simulink model "sys1"  (R2023b)
settings: Solver=VariableStepAuto  StartTime=0.0  StopTime=30e-3  RelTol=1e-3
InitFcn:
  | fs = 100e6;
  | ts = 1 / fs;
values from neighbouring files (symbols this model uses):
  c = 3e8    (= 300000000)    [init_param.m]
  H_az1 = zeros(numSamples,numPulses)    [init_param.m]
  H_az2 = zeros(numSamples,numPulses)    [init_param.m]
  H_ref = fft(conj(fliplr(txChirp)), numSamples)    [init_param.m]
  rawData = rawData + 0.01 * (randn(size(rawData)) + 1j * randn(size(rawData)))    [init_param.m]
  x1 = zeros(size(rawData))    [main.m]
  x2 = zeros(size(x1))    [main.m]
  x3 = zeros(size(x2))    [main.m]
  x4 = zeros(size(x3))    [main.m]
  x5 = zeros(size(x4))    [main.m]
  x6 = zeros(size(x5))    [main.m]
  xx4 = zeros(size(xx3))    [main.m]
  xx5 = zeros(size(xx4))    [main.m]
  xx6 = zeros(size(xx5))    [main.m]
undefined symbols (not defined in the file or in its folder): ffva1156, w2, w3, w4, w5, w6, w7, w8, w9, ww2, ww3, ww4, ww5, ww6, ww7, ww8, ww9, xcku095
libraries: hdlBasic x917, hdlDSPIP x18, dspsrcs4 x12, vmcUtilities x1
(part 4 of 9)

== system sys1/SAR/stream/stream_ifft/stage6 ==
  en : Inport
  re : Inport  Port=2
  im : Inport  Port=3
  BF : Subsystem
      settings: PortSchema="{\"entries\":[{\"content\":{\"sides\":[{\"content\":{\"connectorIds\":[\"In1\",\"In2\",\"Out3\",\"Out4\",\"In3\",\"In4\"]},\"type\":\"ConnectorPlacement.EquallySpacedRectSide\",\"uuid\":\"975bd1ab-81ed-4ae7-b1e2-8f492a85d8f1\"},{\"content\":{\"connectorIds\":[\"Out1\",\"Out2\"],\"side\":\"RIGHT\"},\"type\":\"ConnectorPlacement.EquallySpacedRectSide\",\"uuid\":\"1eadf147-5ad8-47d9-8b00-0d3bf9cf32a8\"},{\"content\":{\"side\":\"TOP\"},\"type\":\"ConnectorPlacement.EquallySpacedRectSide\",\"uuid\":\"8c547c25-4f14-4718-a05d-45e4b8488b96\"}]},\"type\":\"ConnectorPlacement.EquallySpacedConnector\",\"uuid\":\"01bb5c7b-b675-4632-bc6b-a159d4a2e208\"}],\"packageUris\":[\"http://schema.mathworks.com/mf0/Connector/R2020b\"],\"version\":\"1.0\"}"
  Constant : hdlBasic/Constant  const=2^15  gui_display_data_type=Fixed-point  arith_type=Unsigned  n_bits=20  bin_pt=0  preci_type=Single  exp_width=8  frac_width=24  explicit_period=off  period=1  XmcBlockStatus=1  maskContainerNames=tabcontainer1  block_type=constant  block_config=sysgen:Constant_config
  Constant1 : hdlBasic/Constant  const=1  gui_display_data_type=Boolean  arith_type=Boolean  n_bits=16  bin_pt=14  preci_type=Single  exp_width=8  frac_width=24  explicit_period=on  period=ts  XmcBlockStatus=1  maskContainerNames=tabcontainer1  block_type=constant  block_config=sysgen:Constant_config
  Counter1 : hdlBasic/Counter  cnt_type=Free running  cnt_to=Inf  operation=Up  start_count=0  cnt_by_val=1  arith_type=Unsigned  n_bits=20  bin_pt=0  load_pin=off  rst=off  en=on  explicit_period=Explicit  period=ts  use_behavioral_HDL=off  implementation=Fabric  XmcBlockStatus=1  maskContainerNames=group1  block_type=counter  block_config=sysgen:Counter_config  block_width=531  block_height=1023
  Delay11 : hdlBasic/Delay  rst=off  en=off  latency=6  reg_retiming=off  XmcBlockStatus=1  maskContainerNames=group1  block_type=delay  block_config=sysgen:Delay_config
  Delay7 : hdlBasic/Delay  rst=off  en=off  latency=1  reg_retiming=off  XmcBlockStatus=1  maskContainerNames=group1  block_type=delay  block_config=sysgen:Delay_config
  Delay8 : hdlBasic/Delay  rst=off  en=off  latency=1  reg_retiming=off  XmcBlockStatus=1  maskContainerNames=group1  block_type=delay  block_config=sysgen:Delay_config
  Multiplexer : Subsystem
      settings: PortSchema="{\"entries\":[{\"content\":{\"sides\":[{\"content\":{\"connectorIds\":[\"In1\",\"In2\",\"In3\",\"In4\"]},\"type\":\"ConnectorPlacement.EquallySpacedRectSide\",\"uuid\":\"d39b2674-e61f-4632-a918-ea673b128ff5\"},{\"content\":{\"connectorIds\":[\"Out1\",\"Out2\"],\"side\":\"RIGHT\"},\"type\":\"ConnectorPlacement.EquallySpacedRectSide\",\"uuid\":\"03c9bc0a-e0d2-45eb-9b7a-9d06bc1b3e13\"},{\"content\":{\"connectorIds\":[\"In5\"],\"side\":\"TOP\"},\"type\":\"ConnectorPlacement.EquallySpacedRectSide\",\"uuid\":\"49e788e0-ebb0-431e-96ea-edf312796710\"}]},\"type\":\"ConnectorPlacement.EquallySpacedConnector\",\"uuid\":\"eef61444-07bb-4ce5-a4f8-b8563d493c59\"}],\"packageUris\":[\"http://schema.mathworks.com/mf0/Connector/R2020b\"],\"version\":\"1.0\"}"
  Register2 : hdlBasic/Register  init=0  rst=off  en=on  XmcBlockStatus=1  maskContainerNames=tabcontainer1  block_type=register  block_config=sysgen:Register_config
  Relational : hdlBasic/Relational  mode=a=b  op_type=Bool  en=off  latency=0  XmcBlockStatus=1  maskContainerNames=tabcontainer1  block_type=relational  block_config=sysgen:Relational_config
  Shift2 : hdlBasic/Shift  shift_dir=Right  shift_bits=1  en=off  latency=0  precision=User Defined  arith_type="Signed  (2's comp)"  n_bits=16  bin_pt=0  quantization="Round  (unbiased: +/- Inf)"  overflow=Flag as error  XmcBlockStatus=1  maskContainerNames=group2  block_type=shift  block_config=sysgen:Shift_config
  Shift3 : hdlBasic/Shift  shift_dir=Right  shift_bits=1  en=off  latency=0  precision=User Defined  arith_type="Signed  (2's comp)"  n_bits=16  bin_pt=0  quantization="Round  (unbiased: +/- Inf)"  overflow=Flag as error  XmcBlockStatus=1  maskContainerNames=group2  block_type=shift  block_config=sysgen:Shift_config
  Twiddle1 : Subsystem
      settings: PortSchema="{\"entries\":[{\"content\":{\"sides\":[{\"content\":{\"connectorIds\":[\"In1\",\"In2\"]},\"type\":\"ConnectorPlacement.EquallySpacedRectSide\",\"uuid\":\"3a95ef15-fc61-4ad6-8380-7417c0bf925f\"},{\"content\":{\"connectorIds\":[\"Out1\",\"Out2\"],\"side\":\"RIGHT\"},\"type\":\"ConnectorPlacement.EquallySpacedRectSide\",\"uuid\":\"0430fa0d-aaaf-45a9-9ba5-469212780f48\"},{\"content\":{\"connectorIds\":[\"In3\"],\"side\":\"TOP\"},\"type\":\"ConnectorPlacement.EquallySpacedRectSide\",\"uuid\":\"c44a7ed1-335c-4ec2-97d7-9de8a0fe1bfa\"}]},\"type\":\"ConnectorPlacement.EquallySpacedConnector\",\"uuid\":\"1391f0d5-c6a7-4a7e-8f95-f600f2d41ad0\"}],\"packageUris\":[\"http://schema.mathworks.com/mf0/Connector/R2020b\"],\"version\":\"1.0\"}"
  delay : Subsystem
      settings: PortSchema="{\"entries\":[{\"content\":{\"sides\":[{\"content\":{\"connectorIds\":[\"In1\",\"In2\"]},\"type\":\"ConnectorPlacement.EquallySpacedRectSide\",\"uuid\":\"8e95d830-f739-4680-8e8d-a694a3d776c9\"},{\"content\":{\"connectorIds\":[\"Out1\",\"Out2\",\"In4\",\"In5\"],\"side\":\"RIGHT\"},\"type\":\"ConnectorPlacement.EquallySpacedRectSide\",\"uuid\":\"bd1208a8-56cb-479f-9e66-9cf6d0e57587\"},{\"content\":{\"connectorIds\":[\"In3\"],\"side\":\"TOP\"},\"type\":\"ConnectorPlacement.EquallySpacedRectSide\",\"uuid\":\"57cbc148-baa9-4a2d-b86c-5e5c9d420efc\"}]},\"type\":\"ConnectorPlacement.EquallySpacedConnector\",\"uuid\":\"451ef570-de0a-4096-83a7-e8ad0739923f\"}],\"packageUris\":[\"http://schema.mathworks.com/mf0/Connector/R2020b\"],\"version\":\"1.0\"}"
  valid : Outport
  out_re : Outport  Port=2
  out_im : Outport  Port=3
  wires:
  Shift3/1 -> Delay8/1
  Shift2/1 -> Delay7/1
  Constant1/1 -> Register2/1
  Relational/1 -> Register2/2
  Constant/1 -> Relational/2
  re/1 -> Shift2/1
  im/1 -> Shift3/1
  Register2/1 -> Delay11/1
  Counter1/1 -> Multiplexer/5(cnt), Twiddle1/3(cnt), delay/3(cnt), Relational/1
  BF/1(Out2_r) -> Multiplexer/3(r1)
  BF/2(Out2_i) -> Multiplexer/4(i1)
  Twiddle1/2(ii) -> BF/4(vi)
  Twiddle1/1(rr) -> BF/3(vr)
  BF/3(Out1_r) -> delay/4(r1)
  BF/4(Out1_i) -> delay/5(i1)
  delay/1(rr) -> Multiplexer/1(r2), BF/1(ur)
  delay/2(ii) -> Multiplexer/2(i2), BF/2(ui)
  Delay7/1 -> delay/1(r), Twiddle1/1(r)
  Delay8/1 -> delay/2(i), Twiddle1/2(i)
  en/1 -> Counter1/1
  Delay11/1 -> valid/1
  Multiplexer/1(rr) -> out_re/1
  Multiplexer/2(ii) -> out_im/1

== system sys1/SAR/stream/stream_ifft/stage7 ==
  en : Inport
  re : Inport  Port=2
  im : Inport  Port=3
  BF : Subsystem
      settings: PortSchema="{\"entries\":[{\"content\":{\"sides\":[{\"content\":{\"connectorIds\":[\"In1\",\"In2\",\"Out3\",\"Out4\",\"In3\",\"In4\"]},\"type\":\"ConnectorPlacement.EquallySpacedRectSide\",\"uuid\":\"975bd1ab-81ed-4ae7-b1e2-8f492a85d8f1\"},{\"content\":{\"connectorIds\":[\"Out1\",\"Out2\"],\"side\":\"RIGHT\"},\"type\":\"ConnectorPlacement.EquallySpacedRectSide\",\"uuid\":\"1eadf147-5ad8-47d9-8b00-0d3bf9cf32a8\"},{\"content\":{\"side\":\"TOP\"},\"type\":\"ConnectorPlacement.EquallySpacedRectSide\",\"uuid\":\"8c547c25-4f14-4718-a05d-45e4b8488b96\"}]},\"type\":\"ConnectorPlacement.EquallySpacedConnector\",\"uuid\":\"01bb5c7b-b675-4632-bc6b-a159d4a2e208\"}],\"packageUris\":[\"http://schema.mathworks.com/mf0/Connector/R2020b\"],\"version\":\"1.0\"}"
  Constant : hdlBasic/Constant  const=2^16  gui_display_data_type=Fixed-point  arith_type=Unsigned  n_bits=20  bin_pt=0  preci_type=Single  exp_width=8  frac_width=24  explicit_period=off  period=1  XmcBlockStatus=1  maskContainerNames=tabcontainer1  block_type=constant  block_config=sysgen:Constant_config
  Constant1 : hdlBasic/Constant  const=1  gui_display_data_type=Boolean  arith_type=Boolean  n_bits=16  bin_pt=14  preci_type=Single  exp_width=8  frac_width=24  explicit_period=on  period=ts  XmcBlockStatus=1  maskContainerNames=tabcontainer1  block_type=constant  block_config=sysgen:Constant_config
  Counter1 : hdlBasic/Counter  cnt_type=Free running  cnt_to=Inf  operation=Up  start_count=0  cnt_by_val=1  arith_type=Unsigned  n_bits=20  bin_pt=0  load_pin=off  rst=off  en=on  explicit_period=Explicit  period=ts  use_behavioral_HDL=off  implementation=Fabric  XmcBlockStatus=1  maskContainerNames=group1  block_type=counter  block_config=sysgen:Counter_config  block_width=531  block_height=1023
  Delay11 : hdlBasic/Delay  rst=off  en=off  latency=6  reg_retiming=off  XmcBlockStatus=1  maskContainerNames=group1  block_type=delay  block_config=sysgen:Delay_config
  Delay7 : hdlBasic/Delay  rst=off  en=off  latency=1  reg_retiming=off  XmcBlockStatus=1  maskContainerNames=group1  block_type=delay  block_config=sysgen:Delay_config
  Delay8 : hdlBasic/Delay  rst=off  en=off  latency=1  reg_retiming=off  XmcBlockStatus=1  maskContainerNames=group1  block_type=delay  block_config=sysgen:Delay_config
  Multiplexer : Subsystem
      settings: PortSchema="{\"entries\":[{\"content\":{\"sides\":[{\"content\":{\"connectorIds\":[\"In1\",\"In2\",\"In3\",\"In4\"]},\"type\":\"ConnectorPlacement.EquallySpacedRectSide\",\"uuid\":\"d39b2674-e61f-4632-a918-ea673b128ff5\"},{\"content\":{\"connectorIds\":[\"Out1\",\"Out2\"],\"side\":\"RIGHT\"},\"type\":\"ConnectorPlacement.EquallySpacedRectSide\",\"uuid\":\"03c9bc0a-e0d2-45eb-9b7a-9d06bc1b3e13\"},{\"content\":{\"connectorIds\":[\"In5\"],\"side\":\"TOP\"},\"type\":\"ConnectorPlacement.EquallySpacedRectSide\",\"uuid\":\"49e788e0-ebb0-431e-96ea-edf312796710\"}]},\"type\":\"ConnectorPlacement.EquallySpacedConnector\",\"uuid\":\"eef61444-07bb-4ce5-a4f8-b8563d493c59\"}],\"packageUris\":[\"http://schema.mathworks.com/mf0/Connector/R2020b\"],\"version\":\"1.0\"}"
  Register2 : hdlBasic/Register  init=0  rst=off  en=on  XmcBlockStatus=1  maskContainerNames=tabcontainer1  block_type=register  block_config=sysgen:Register_config
  Relational : hdlBasic/Relational  mode=a=b  op_type=Bool  en=off  latency=0  XmcBlockStatus=1  maskContainerNames=tabcontainer1  block_type=relational  block_config=sysgen:Relational_config
  Shift2 : hdlBasic/Shift  shift_dir=Right  shift_bits=1  en=off  latency=0  precision=User Defined  arith_type="Signed  (2's comp)"  n_bits=16  bin_pt=0  quantization="Round  (unbiased: +/- Inf)"  overflow=Flag as error  XmcBlockStatus=1  maskContainerNames=group2  block_type=shift  block_config=sysgen:Shift_config
  Shift3 : hdlBasic/Shift  shift_dir=Right  shift_bits=1  en=off  latency=0  precision=User Defined  arith_type="Signed  (2's comp)"  n_bits=16  bin_pt=0  quantization="Round  (unbiased: +/- Inf)"  overflow=Flag as error  XmcBlockStatus=1  maskContainerNames=group2  block_type=shift  block_config=sysgen:Shift_config
  Twiddle1 : Subsystem
      settings: PortSchema="{\"entries\":[{\"content\":{\"sides\":[{\"content\":{\"connectorIds\":[\"In1\",\"In2\"]},\"type\":\"ConnectorPlacement.EquallySpacedRectSide\",\"uuid\":\"3a95ef15-fc61-4ad6-8380-7417c0bf925f\"},{\"content\":{\"connectorIds\":[\"Out1\",\"Out2\"],\"side\":\"RIGHT\"},\"type\":\"ConnectorPlacement.EquallySpacedRectSide\",\"uuid\":\"0430fa0d-aaaf-45a9-9ba5-469212780f48\"},{\"content\":{\"connectorIds\":[\"In3\"],\"side\":\"TOP\"},\"type\":\"ConnectorPlacement.EquallySpacedRectSide\",\"uuid\":\"c44a7ed1-335c-4ec2-97d7-9de8a0fe1bfa\"}]},\"type\":\"ConnectorPlacement.EquallySpacedConnector\",\"uuid\":\"1391f0d5-c6a7-4a7e-8f95-f600f2d41ad0\"}],\"packageUris\":[\"http://schema.mathworks.com/mf0/Connector/R2020b\"],\"version\":\"1.0\"}"
  delay : Subsystem
      settings: PortSchema="{\"entries\":[{\"content\":{\"sides\":[{\"content\":{\"connectorIds\":[\"In1\",\"In2\"]},\"type\":\"ConnectorPlacement.EquallySpacedRectSide\",\"uuid\":\"8e95d830-f739-4680-8e8d-a694a3d776c9\"},{\"content\":{\"connectorIds\":[\"Out1\",\"Out2\",\"In4\",\"In5\"],\"side\":\"RIGHT\"},\"type\":\"ConnectorPlacement.EquallySpacedRectSide\",\"uuid\":\"bd1208a8-56cb-479f-9e66-9cf6d0e57587\"},{\"content\":{\"connectorIds\":[\"In3\"],\"side\":\"TOP\"},\"type\":\"ConnectorPlacement.EquallySpacedRectSide\",\"uuid\":\"57cbc148-baa9-4a2d-b86c-5e5c9d420efc\"}]},\"type\":\"ConnectorPlacement.EquallySpacedConnector\",\"uuid\":\"451ef570-de0a-4096-83a7-e8ad0739923f\"}],\"packageUris\":[\"http://schema.mathworks.com/mf0/Connector/R2020b\"],\"version\":\"1.0\"}"
  valid : Outport
  out_re : Outport  Port=2
  out_im : Outport  Port=3
  wires:
  Shift3/1 -> Delay8/1
  Shift2/1 -> Delay7/1
  Delay11/1 -> valid/1
  en/1 -> Counter1/1
  Delay8/1 -> Twiddle1/2(i), delay/2(i)
  Delay7/1 -> Twiddle1/1(r), delay/1(r)
  delay/2(ii) -> Multiplexer/2(i2), BF/2(ui)
  delay/1(rr) -> Multiplexer/1(r2), BF/1(ur)
  BF/4(Out1_i) -> delay/5(i1)
  BF/3(Out1_r) -> delay/4(r1)
  Twiddle1/1(rr) -> BF/3(vr)
  Twiddle1/2(ii) -> BF/4(vi)
  BF/2(Out2_i) -> Multiplexer/4(i1)
  BF/1(Out2_r) -> Multiplexer/3(r1)
  Counter1/1 -> Relational/1, delay/3(cnt), Twiddle1/3(cnt), Multiplexer/5(cnt)
  Register2/1 -> Delay11/1
  im/1 -> Shift3/1
  re/1 -> Shift2/1
  Constant/1 -> Relational/2
  Relational/1 -> Register2/2
  Constant1/1 -> Register2/1
  Multiplexer/1(rr) -> out_re/1
  Multiplexer/2(ii) -> out_im/1

== system sys1/SAR/stream/stream_ifft/stage8 ==
  en : Inport
  re : Inport  Port=2
  im : Inport  Port=3
  BF : Subsystem
      settings: PortSchema="{\"entries\":[{\"content\":{\"sides\":[{\"content\":{\"connectorIds\":[\"In1\",\"In2\",\"Out3\",\"Out4\",\"In3\",\"In4\"]},\"type\":\"ConnectorPlacement.EquallySpacedRectSide\",\"uuid\":\"975bd1ab-81ed-4ae7-b1e2-8f492a85d8f1\"},{\"content\":{\"connectorIds\":[\"Out1\",\"Out2\"],\"side\":\"RIGHT\"},\"type\":\"ConnectorPlacement.EquallySpacedRectSide\",\"uuid\":\"1eadf147-5ad8-47d9-8b00-0d3bf9cf32a8\"},{\"content\":{\"side\":\"TOP\"},\"type\":\"ConnectorPlacement.EquallySpacedRectSide\",\"uuid\":\"8c547c25-4f14-4718-a05d-45e4b8488b96\"}]},\"type\":\"ConnectorPlacement.EquallySpacedConnector\",\"uuid\":\"01bb5c7b-b675-4632-bc6b-a159d4a2e208\"}],\"packageUris\":[\"http://schema.mathworks.com/mf0/Connector/R2020b\"],\"version\":\"1.0\"}"
  Constant : hdlBasic/Constant  const=2^17  gui_display_data_type=Fixed-point  arith_type=Unsigned  n_bits=20  bin_pt=0  preci_type=Single  exp_width=8  frac_width=24  explicit_period=off  period=1  XmcBlockStatus=1  maskContainerNames=tabcontainer1  block_type=constant  block_config=sysgen:Constant_config
  Constant1 : hdlBasic/Constant  const=1  gui_display_data_type=Boolean  arith_type=Boolean  n_bits=16  bin_pt=14  preci_type=Single  exp_width=8  frac_width=24  explicit_period=on  period=ts  XmcBlockStatus=1  maskContainerNames=tabcontainer1  block_type=constant  block_config=sysgen:Constant_config
  Counter1 : hdlBasic/Counter  cnt_type=Free running  cnt_to=Inf  operation=Up  start_count=0  cnt_by_val=1  arith_type=Unsigned  n_bits=20  bin_pt=0  load_pin=off  rst=off  en=on  explicit_period=Explicit  period=ts  use_behavioral_HDL=off  implementation=Fabric  XmcBlockStatus=1  maskContainerNames=group1  block_type=counter  block_config=sysgen:Counter_config  block_width=531  block_height=1023
  Delay11 : hdlBasic/Delay  rst=off  en=off  latency=6  reg_retiming=off  XmcBlockStatus=1  maskContainerNames=group1  block_type=delay  block_config=sysgen:Delay_config
  Delay7 : hdlBasic/Delay  rst=off  en=off  latency=1  reg_retiming=off  XmcBlockStatus=1  maskContainerNames=group1  block_type=delay  block_config=sysgen:Delay_config
  Delay8 : hdlBasic/Delay  rst=off  en=off  latency=1  reg_retiming=off  XmcBlockStatus=1  maskContainerNames=group1  block_type=delay  block_config=sysgen:Delay_config
  Multiplexer : Subsystem
      settings: PortSchema="{\"entries\":[{\"content\":{\"sides\":[{\"content\":{\"connectorIds\":[\"In1\",\"In2\",\"In3\",\"In4\"]},\"type\":\"ConnectorPlacement.EquallySpacedRectSide\",\"uuid\":\"d39b2674-e61f-4632-a918-ea673b128ff5\"},{\"content\":{\"connectorIds\":[\"Out1\",\"Out2\"],\"side\":\"RIGHT\"},\"type\":\"ConnectorPlacement.EquallySpacedRectSide\",\"uuid\":\"03c9bc0a-e0d2-45eb-9b7a-9d06bc1b3e13\"},{\"content\":{\"connectorIds\":[\"In5\"],\"side\":\"TOP\"},\"type\":\"ConnectorPlacement.EquallySpacedRectSide\",\"uuid\":\"49e788e0-ebb0-431e-96ea-edf312796710\"}]},\"type\":\"ConnectorPlacement.EquallySpacedConnector\",\"uuid\":\"eef61444-07bb-4ce5-a4f8-b8563d493c59\"}],\"packageUris\":[\"http://schema.mathworks.com/mf0/Connector/R2020b\"],\"version\":\"1.0\"}"
  Register2 : hdlBasic/Register  init=0  rst=off  en=on  XmcBlockStatus=1  maskContainerNames=tabcontainer1  block_type=register  block_config=sysgen:Register_config
  Relational : hdlBasic/Relational  mode=a=b  op_type=Bool  en=off  latency=0  XmcBlockStatus=1  maskContainerNames=tabcontainer1  block_type=relational  block_config=sysgen:Relational_config
  Shift2 : hdlBasic/Shift  shift_dir=Right  shift_bits=1  en=off  latency=0  precision=User Defined  arith_type="Signed  (2's comp)"  n_bits=16  bin_pt=0  quantization="Round  (unbiased: +/- Inf)"  overflow=Flag as error  XmcBlockStatus=1  maskContainerNames=group2  block_type=shift  block_config=sysgen:Shift_config
  Shift3 : hdlBasic/Shift  shift_dir=Right  shift_bits=1  en=off  latency=0  precision=User Defined  arith_type="Signed  (2's comp)"  n_bits=16  bin_pt=0  quantization="Round  (unbiased: +/- Inf)"  overflow=Flag as error  XmcBlockStatus=1  maskContainerNames=group2  block_type=shift  block_config=sysgen:Shift_config
  Twiddle1 : Subsystem
      settings: PortSchema="{\"entries\":[{\"content\":{\"sides\":[{\"content\":{\"connectorIds\":[\"In1\",\"In2\"]},\"type\":\"ConnectorPlacement.EquallySpacedRectSide\",\"uuid\":\"3a95ef15-fc61-4ad6-8380-7417c0bf925f\"},{\"content\":{\"connectorIds\":[\"Out1\",\"Out2\"],\"side\":\"RIGHT\"},\"type\":\"ConnectorPlacement.EquallySpacedRectSide\",\"uuid\":\"0430fa0d-aaaf-45a9-9ba5-469212780f48\"},{\"content\":{\"connectorIds\":[\"In3\"],\"side\":\"TOP\"},\"type\":\"ConnectorPlacement.EquallySpacedRectSide\",\"uuid\":\"c44a7ed1-335c-4ec2-97d7-9de8a0fe1bfa\"}]},\"type\":\"ConnectorPlacement.EquallySpacedConnector\",\"uuid\":\"1391f0d5-c6a7-4a7e-8f95-f600f2d41ad0\"}],\"packageUris\":[\"http://schema.mathworks.com/mf0/Connector/R2020b\"],\"version\":\"1.0\"}"
  delay : Subsystem
      settings: PortSchema="{\"entries\":[{\"content\":{\"sides\":[{\"content\":{\"connectorIds\":[\"In1\",\"In2\"]},\"type\":\"ConnectorPlacement.EquallySpacedRectSide\",\"uuid\":\"8e95d830-f739-4680-8e8d-a694a3d776c9\"},{\"content\":{\"connectorIds\":[\"Out1\",\"Out2\",\"In4\",\"In5\"],\"side\":\"RIGHT\"},\"type\":\"ConnectorPlacement.EquallySpacedRectSide\",\"uuid\":\"bd1208a8-56cb-479f-9e66-9cf6d0e57587\"},{\"content\":{\"connectorIds\":[\"In3\"],\"side\":\"TOP\"},\"type\":\"ConnectorPlacement.EquallySpacedRectSide\",\"uuid\":\"57cbc148-baa9-4a2d-b86c-5e5c9d420efc\"}]},\"type\":\"ConnectorPlacement.EquallySpacedConnector\",\"uuid\":\"451ef570-de0a-4096-83a7-e8ad0739923f\"}],\"packageUris\":[\"http://schema.mathworks.com/mf0/Connector/R2020b\"],\"version\":\"1.0\"}"
  valid : Outport
  out_re : Outport  Port=2
  out_im : Outport  Port=3
  wires:
  Shift3/1 -> Delay8/1
  Shift2/1 -> Delay7/1
  Constant1/1 -> Register2/1
  Relational/1 -> Register2/2
  Constant/1 -> Relational/2
  re/1 -> Shift2/1
  im/1 -> Shift3/1
  Register2/1 -> Delay11/1
  Counter1/1 -> Multiplexer/5(cnt), Twiddle1/3(cnt), delay/3(cnt), Relational/1
  BF/1(Out2_r) -> Multiplexer/3(r1)
  BF/2(Out2_i) -> Multiplexer/4(i1)
  Twiddle1/2(ii) -> BF/4(vi)
  Twiddle1/1(rr) -> BF/3(vr)
  BF/3(Out1_r) -> delay/4(r1)
  BF/4(Out1_i) -> delay/5(i1)
  delay/1(rr) -> Multiplexer/1(r2), BF/1(ur)
  delay/2(ii) -> Multiplexer/2(i2), BF/2(ui)
  Delay7/1 -> delay/1(r), Twiddle1/1(r)
  Delay8/1 -> delay/2(i), Twiddle1/2(i)
  en/1 -> Counter1/1
  Delay11/1 -> valid/1
  Multiplexer/1(rr) -> out_re/1
  Multiplexer/2(ii) -> out_im/1

== system sys1/SAR/stream/stream_ifft/stage9 ==
  en : Inport
  re : Inport  Port=2
  im : Inport  Port=3
  BF : Subsystem
      settings: PortSchema="{\"entries\":[{\"content\":{\"sides\":[{\"content\":{\"connectorIds\":[\"In1\",\"In2\",\"Out3\",\"Out4\",\"In3\",\"In4\"]},\"type\":\"ConnectorPlacement.EquallySpacedRectSide\",\"uuid\":\"975bd1ab-81ed-4ae7-b1e2-8f492a85d8f1\"},{\"content\":{\"connectorIds\":[\"Out1\",\"Out2\"],\"side\":\"RIGHT\"},\"type\":\"ConnectorPlacement.EquallySpacedRectSide\",\"uuid\":\"1eadf147-5ad8-47d9-8b00-0d3bf9cf32a8\"},{\"content\":{\"side\":\"TOP\"},\"type\":\"ConnectorPlacement.EquallySpacedRectSide\",\"uuid\":\"8c547c25-4f14-4718-a05d-45e4b8488b96\"}]},\"type\":\"ConnectorPlacement.EquallySpacedConnector\",\"uuid\":\"01bb5c7b-b675-4632-bc6b-a159d4a2e208\"}],\"packageUris\":[\"http://schema.mathworks.com/mf0/Connector/R2020b\"],\"version\":\"1.0\"}"
  Constant : hdlBasic/Constant  const=2^18  gui_display_data_type=Fixed-point  arith_type=Unsigned  n_bits=20  bin_pt=0  preci_type=Single  exp_width=8  frac_width=24  explicit_period=off  period=1  XmcBlockStatus=1  maskContainerNames=tabcontainer1  block_type=constant  block_config=sysgen:Constant_config
  Constant1 : hdlBasic/Constant  const=1  gui_display_data_type=Boolean  arith_type=Boolean  n_bits=16  bin_pt=14  preci_type=Single  exp_width=8  frac_width=24  explicit_period=on  period=ts  XmcBlockStatus=1  maskContainerNames=tabcontainer1  block_type=constant  block_config=sysgen:Constant_config
  Counter1 : hdlBasic/Counter  cnt_type=Free running  cnt_to=Inf  operation=Up  start_count=0  cnt_by_val=1  arith_type=Unsigned  n_bits=20  bin_pt=0  load_pin=off  rst=off  en=on  explicit_period=Explicit  period=ts  use_behavioral_HDL=off  implementation=Fabric  XmcBlockStatus=1  maskContainerNames=group1  block_type=counter  block_config=sysgen:Counter_config  block_width=531  block_height=1023
  Delay11 : hdlBasic/Delay  rst=off  en=off  latency=6  reg_retiming=off  XmcBlockStatus=1  maskContainerNames=group1  block_type=delay  block_config=sysgen:Delay_config
  Delay7 : hdlBasic/Delay  rst=off  en=off  latency=1  reg_retiming=off  XmcBlockStatus=1  maskContainerNames=group1  block_type=delay  block_config=sysgen:Delay_config
  Delay8 : hdlBasic/Delay  rst=off  en=off  latency=1  reg_retiming=off  XmcBlockStatus=1  maskContainerNames=group1  block_type=delay  block_config=sysgen:Delay_config
  Multiplexer : Subsystem
      settings: PortSchema="{\"entries\":[{\"content\":{\"sides\":[{\"content\":{\"connectorIds\":[\"In1\",\"In2\",\"In3\",\"In4\"]},\"type\":\"ConnectorPlacement.EquallySpacedRectSide\",\"uuid\":\"d39b2674-e61f-4632-a918-ea673b128ff5\"},{\"content\":{\"connectorIds\":[\"Out1\",\"Out2\"],\"side\":\"RIGHT\"},\"type\":\"ConnectorPlacement.EquallySpacedRectSide\",\"uuid\":\"03c9bc0a-e0d2-45eb-9b7a-9d06bc1b3e13\"},{\"content\":{\"connectorIds\":[\"In5\"],\"side\":\"TOP\"},\"type\":\"ConnectorPlacement.EquallySpacedRectSide\",\"uuid\":\"49e788e0-ebb0-431e-96ea-edf312796710\"}]},\"type\":\"ConnectorPlacement.EquallySpacedConnector\",\"uuid\":\"eef61444-07bb-4ce5-a4f8-b8563d493c59\"}],\"packageUris\":[\"http://schema.mathworks.com/mf0/Connector/R2020b\"],\"version\":\"1.0\"}"
  Register2 : hdlBasic/Register  init=0  rst=off  en=on  XmcBlockStatus=1  maskContainerNames=tabcontainer1  block_type=register  block_config=sysgen:Register_config
  Relational : hdlBasic/Relational  mode=a=b  op_type=Bool  en=off  latency=0  XmcBlockStatus=1  maskContainerNames=tabcontainer1  block_type=relational  block_config=sysgen:Relational_config
  Shift2 : hdlBasic/Shift  shift_dir=Right  shift_bits=1  en=off  latency=0  precision=User Defined  arith_type="Signed  (2's comp)"  n_bits=16  bin_pt=0  quantization="Round  (unbiased: +/- Inf)"  overflow=Flag as error  XmcBlockStatus=1  maskContainerNames=group2  block_type=shift  block_config=sysgen:Shift_config
  Shift3 : hdlBasic/Shift  shift_dir=Right  shift_bits=1  en=off  latency=0  precision=User Defined  arith_type="Signed  (2's comp)"  n_bits=16  bin_pt=0  quantization="Round  (unbiased: +/- Inf)"  overflow=Flag as error  XmcBlockStatus=1  maskContainerNames=group2  block_type=shift  block_config=sysgen:Shift_config
  Twiddle1 : Subsystem
      settings: PortSchema="{\"entries\":[{\"content\":{\"sides\":[{\"content\":{\"connectorIds\":[\"In1\",\"In2\"]},\"type\":\"ConnectorPlacement.EquallySpacedRectSide\",\"uuid\":\"3a95ef15-fc61-4ad6-8380-7417c0bf925f\"},{\"content\":{\"connectorIds\":[\"Out1\",\"Out2\"],\"side\":\"RIGHT\"},\"type\":\"ConnectorPlacement.EquallySpacedRectSide\",\"uuid\":\"0430fa0d-aaaf-45a9-9ba5-469212780f48\"},{\"content\":{\"connectorIds\":[\"In3\"],\"side\":\"TOP\"},\"type\":\"ConnectorPlacement.EquallySpacedRectSide\",\"uuid\":\"c44a7ed1-335c-4ec2-97d7-9de8a0fe1bfa\"}]},\"type\":\"ConnectorPlacement.EquallySpacedConnector\",\"uuid\":\"1391f0d5-c6a7-4a7e-8f95-f600f2d41ad0\"}],\"packageUris\":[\"http://schema.mathworks.com/mf0/Connector/R2020b\"],\"version\":\"1.0\"}"
  delay : Subsystem
      settings: PortSchema="{\"entries\":[{\"content\":{\"sides\":[{\"content\":{\"connectorIds\":[\"In1\",\"In2\"]},\"type\":\"ConnectorPlacement.EquallySpacedRectSide\",\"uuid\":\"8e95d830-f739-4680-8e8d-a694a3d776c9\"},{\"content\":{\"connectorIds\":[\"Out1\",\"Out2\",\"In4\",\"In5\"],\"side\":\"RIGHT\"},\"type\":\"ConnectorPlacement.EquallySpacedRectSide\",\"uuid\":\"bd1208a8-56cb-479f-9e66-9cf6d0e57587\"},{\"content\":{\"connectorIds\":[\"In3\"],\"side\":\"TOP\"},\"type\":\"ConnectorPlacement.EquallySpacedRectSide\",\"uuid\":\"57cbc148-baa9-4a2d-b86c-5e5c9d420efc\"}]},\"type\":\"ConnectorPlacement.EquallySpacedConnector\",\"uuid\":\"451ef570-de0a-4096-83a7-e8ad0739923f\"}],\"packageUris\":[\"http://schema.mathworks.com/mf0/Connector/R2020b\"],\"version\":\"1.0\"}"
  valid : Outport
  out_re : Outport  Port=2
  out_im : Outport  Port=3
  wires:
  Shift3/1 -> Delay8/1
  Shift2/1 -> Delay7/1
  Delay11/1 -> valid/1
  en/1 -> Counter1/1
  Delay8/1 -> Twiddle1/2(i), delay/2(i)
  Delay7/1 -> Twiddle1/1(r), delay/1(r)
  delay/2(ii) -> Multiplexer/2(i2), BF/2(ui)
  delay/1(rr) -> Multiplexer/1(r2), BF/1(ur)
  BF/4(Out1_i) -> delay/5(i1)
  BF/3(Out1_r) -> delay/4(r1)
  Twiddle1/1(rr) -> BF/3(vr)
  Twiddle1/2(ii) -> BF/4(vi)
  BF/2(Out2_i) -> Multiplexer/4(i1)
  BF/1(Out2_r) -> Multiplexer/3(r1)
  Counter1/1 -> Relational/1, delay/3(cnt), Twiddle1/3(cnt), Multiplexer/5(cnt)
  Register2/1 -> Delay11/1
  im/1 -> Shift3/1
  re/1 -> Shift2/1
  Constant/1 -> Relational/2
  Relational/1 -> Register2/2
  Constant1/1 -> Register2/1
  Multiplexer/1(rr) -> out_re/1
  Multiplexer/2(ii) -> out_im/1

== system sys1/SAR/stream/stream_fft/stage1/BF ==
  re2 : Inport
  im2 : Inport  Port=2
  re1 : Inport  Port=3
  im1 : Inport  Port=4
  AddSub1 : hdlBasic/AddSub  mode=Addition  use_carryin=off  use_carryout=off  en=off  latency=0  precision=User Defined  arith_type="Signed  (2's comp)"  n_bits=16  bin_pt=0  quantization="Round  (unbiased: +/- Inf)"  overflow=Flag as error  use_behavioral_HDL=off  hw_selection=Fabric  pipelined=off  XmcBlockStatus=1  maskContainerNames=tabcontainer1  block_type=addsub  block_config=sysgen:Addsub_config
  AddSub2 : hdlBasic/AddSub  mode=Addition  use_carryin=off  use_carryout=off  en=off  latency=0  precision=User Defined  arith_type="Signed  (2's comp)"  n_bits=16  bin_pt=0  quantization="Round  (unbiased: +/- Inf)"  overflow=Flag as error  use_behavioral_HDL=off  hw_selection=Fabric  pipelined=off  XmcBlockStatus=1  maskContainerNames=tabcontainer1  block_type=addsub  block_config=sysgen:Addsub_config
  AddSub3 : hdlBasic/AddSub  mode=Subtraction  use_carryin=off  use_carryout=off  en=off  latency=0  precision=User Defined  arith_type="Signed  (2's comp)"  n_bits=16  bin_pt=0  quantization="Round  (unbiased: +/- Inf)"  overflow=Flag as error  use_behavioral_HDL=off  hw_selection=Fabric  pipelined=off  XmcBlockStatus=1  maskContainerNames=tabcontainer1  block_type=addsub  block_config=sysgen:Addsub_config
  AddSub4 : hdlBasic/AddSub  mode=Subtraction  use_carryin=off  use_carryout=off  en=off  latency=0  precision=User Defined  arith_type="Signed  (2's comp)"  n_bits=16  bin_pt=0  quantization="Round  (unbiased: +/- Inf)"  overflow=Flag as error  use_behavioral_HDL=off  hw_selection=Fabric  pipelined=off  XmcBlockStatus=1  maskContainerNames=tabcontainer1  block_type=addsub  block_config=sysgen:Addsub_config
  Delay2 : hdlBasic/Delay  rst=off  en=off  latency=7  reg_retiming=off  XmcBlockStatus=1  maskContainerNames=group1  block_type=delay  block_config=sysgen:Delay_config
  Delay3 : hdlBasic/Delay  rst=off  en=off  latency=7  reg_retiming=off  XmcBlockStatus=1  maskContainerNames=group1  block_type=delay  block_config=sysgen:Delay_config
  Out2_r : Outport
  Out2_i : Outport  Port=2
  Out1_r : Outport  Port=3
  Out1_i : Outport  Port=4
  wires:
  AddSub4/1 -> Out1_r/1
  AddSub3/1 -> Out1_i/1
  re2/1 -> AddSub2/1, AddSub4/1
  im2/1 -> AddSub1/1, AddSub3/1
  AddSub2/1 -> Delay2/1
  AddSub1/1 -> Delay3/1
  re1/1 -> AddSub2/2, AddSub4/2
  im1/1 -> AddSub1/2, AddSub3/2
  Delay2/1 -> Out2_r/1
  Delay3/1 -> Out2_i/1

== system sys1/SAR/stream/stream_fft/stage1/Multiplexer ==
  r1 : Inport
  i1 : Inport  Port=2
  r2 : Inport  Port=3
  i2 : Inport  Port=4
  cnt : Inport  Port=5
  BitBasher : hdlBasic/BitBasher  bitexpr=a={b[10]}  display_expr=off  sr_1=a  arith_type1=Unsigned  bin_pt1=0  sr_2=2  arith_type2=Unsigned  bin_pt2=0  sr_3=3  arith_type3=Unsigned  bin_pt3=0  sr_4=4  arith_type4=Unsigned  bin_pt4=0  XmcBlockStatus=1  maskContainerNames=group1  block_type=bitbasher  block_config=sysgen:BitBasher_config
  Inverter : hdlBasic/Inverter  en=off  latency=0  XmcBlockStatus=1  maskContainerNames=group2  block_type=inv  block_config=sysgen:Inverter_config
  Mux : hdlBasic/Mux  inputs=2  en=off  latency=0  precision=Full  arith_type=Unsigned  n_bits=16  bin_pt=14  quantization=Truncate  overflow=Wrap  XmcBlockStatus=1  maskContainerNames=tabcontainer1  block_type=mux  block_config=sysgen:Mux_config
  Mux1 : hdlBasic/Mux  inputs=2  en=off  latency=0  precision=Full  arith_type=Unsigned  n_bits=16  bin_pt=14  quantization=Truncate  overflow=Wrap  XmcBlockStatus=1  maskContainerNames=tabcontainer1  block_type=mux  block_config=sysgen:Mux_config
  rr : Outport
  ii : Outport  Port=2
  wires:
  r1/1 -> Mux/3
  i2/1 -> Mux1/2
  BitBasher/1 -> Inverter/1
  r2/1 -> Mux/2
  i1/1 -> Mux1/3
  Mux1/1 -> ii/1
  Mux/1 -> rr/1
  cnt/1 -> BitBasher/1
  Inverter/1 -> Mux/1, Mux1/1

== system sys1/SAR/stream/stream_fft/stage1/Twiddle ==
  r : Inport
  i : Inport  Port=2
  cnt : Inport  Port=3
  BitBasher1 : hdlBasic/BitBasher  bitexpr=a={b[10:10]}  display_expr=off  sr_1=a  arith_type1=Unsigned  bin_pt1=0  sr_2=2  arith_type2=Unsigned  bin_pt2=0  sr_3=3  arith_type3=Unsigned  bin_pt3=0  sr_4=4  arith_type4=Unsigned  bin_pt4=0  XmcBlockStatus=1  maskContainerNames=group1  block_type=bitbasher  block_config=sysgen:BitBasher_config
  Convert1 : hdlBasic/Convert  gui_display_data_type=Fixed-point  arith_type=Signed (2's comp)  n_bits=16  bin_pt=0  float_type=Single  exp_bits=8  fraction_bits=24  quantization=Truncate  overflow=Flag as error  en=off  latency=0  pipeline=off  XmcBlockStatus=1  maskContainerNames=group2  block_type=convert  block_config=sysgen:Convert_config  block_width=595  block_height=885
  Convert2 : hdlBasic/Convert  gui_display_data_type=Fixed-point  arith_type=Signed (2's comp)  n_bits=16  bin_pt=0  float_type=Single  exp_bits=8  fraction_bits=24  quantization=Truncate  overflow=Flag as error  en=off  latency=0  pipeline=off  XmcBlockStatus=1  maskContainerNames=group2  block_type=convert  block_config=sysgen:Convert_config  block_width=595  block_height=885
  Delay1 : hdlBasic/Delay  rst=off  en=off  latency=6  reg_retiming=off  XmcBlockStatus=1  maskContainerNames=group1  block_type=delay  block_config=sysgen:Delay_config
  Delay2 : hdlBasic/Delay  rst=off  en=off  latency=1  reg_retiming=off  XmcBlockStatus=1  maskContainerNames=group1  block_type=delay  block_config=sysgen:Delay_config
  Delay3 : hdlBasic/Delay  rst=off  en=off  latency=1  reg_retiming=off  XmcBlockStatus=1  maskContainerNames=group1  block_type=delay  block_config=sysgen:Delay_config
  Delay4 : hdlBasic/Delay  rst=off  en=off  latency=6  reg_retiming=off  XmcBlockStatus=1  maskContainerNames=group1  block_type=delay  block_config=sysgen:Delay_config
  ROM : hdlBasic/ROM  depth=length(w2)  initVector=real(w2)  distributed_mem=Block RAM  rst=off  init_reg=0  en=off  latency=1  gui_display_data_type=Fixed-point  arith_type="Signed  (2's comp)"  n_bits=16  bin_pt=15  preci_type=Single  exp_width=8  frac_width=24  optimize=Area  use_rpm=on  simulation_type=fast_sim  XmcBlockStatus=1  maskContainerNames=tabcontainer1  block_type=sprom  block_config=sysgen:SPROM_config
  ROM1 : hdlBasic/ROM  depth=length(w2)  initVector=imag(w2)  distributed_mem=Block RAM  rst=off  init_reg=0  en=off  latency=1  gui_display_data_type=Fixed-point  arith_type="Signed  (2's comp)"  n_bits=16  bin_pt=15  preci_type=Single  exp_width=8  frac_width=24  optimize=Area  use_rpm=on  simulation_type=fast_sim  XmcBlockStatus=1  maskContainerNames=tabcontainer1  block_type=sprom  block_config=sysgen:SPROM_config
  rr : Outport
  ii : Outport  Port=2
  wires:
  BitBasher1/1 -> ROM/1, ROM1/1
  Delay1/1 -> Convert2/1
  i/1 -> Delay2/1
  Delay4/1 -> Convert1/1
  r/1 -> Delay3/1
  cnt/1 -> BitBasher1/1
  Convert2/1 -> ii/1
  Convert1/1 -> rr/1
  Delay2/1 -> Delay1/1
  Delay3/1 -> Delay4/1

== system sys1/SAR/stream/stream_fft/stage1/delay ==
  r : Inport
  i : Inport  Port=2
  cnt : Inport  Port=3
  r1 : Inport  Port=4
  i1 : Inport  Port=5
  BitBasher : hdlBasic/BitBasher  bitexpr=a={b[10]}  display_expr=off  sr_1=a  arith_type1=Unsigned  bin_pt1=0  sr_2=2  arith_type2=Unsigned  bin_pt2=0  sr_3=3  arith_type3=Unsigned  bin_pt3=0  sr_4=4  arith_type4=Unsigned  bin_pt4=0  XmcBlockStatus=1  maskContainerNames=group1  block_type=bitbasher  block_config=sysgen:BitBasher_config
  Inverter : hdlBasic/Inverter  en=off  latency=0  XmcBlockStatus=1  maskContainerNames=group2  block_type=inv  block_config=sysgen:Inverter_config
  Mux : hdlBasic/Mux  inputs=2  en=off  latency=0  precision=Full  arith_type=Unsigned  n_bits=16  bin_pt=14  quantization=Truncate  overflow=Wrap  XmcBlockStatus=1  maskContainerNames=tabcontainer1  block_type=mux  block_config=sysgen:Mux_config
  Mux1 : hdlBasic/Mux  inputs=2  en=off  latency=0  precision=Full  arith_type=Unsigned  n_bits=16  bin_pt=14  quantization=Truncate  overflow=Wrap  XmcBlockStatus=1  maskContainerNames=tabcontainer1  block_type=mux  block_config=sysgen:Mux_config
  delay : Subsystem
  delay1 : Subsystem
  rr : Outport
  ii : Outport  Port=2
  wires:
  Inverter/1 -> Mux1/1, Mux/1
  cnt/1 -> BitBasher/1
  BitBasher/1 -> Inverter/1
  Mux/1 -> delay/1(in)
  Mux1/1 -> delay1/1(in)
  r1/1 -> Mux/2
  i1/1 -> Mux1/2
  delay/1(out) -> rr/1
  delay1/1(out) -> ii/1
  r/1 -> Mux/3
  i/1 -> Mux1/3

== system sys1/SAR/stream/stream_fft/stage2/BF ==
  re2 : Inport
  im2 : Inport  Port=2
  re1 : Inport  Port=3
  im1 : Inport  Port=4
  AddSub1 : hdlBasic/AddSub  mode=Addition  use_carryin=off  use_carryout=off  en=off  latency=0  precision=User Defined  arith_type="Signed  (2's comp)"  n_bits=16  bin_pt=0  quantization="Round  (unbiased: +/- Inf)"  overflow=Flag as error  use_behavioral_HDL=off  hw_selection=Fabric  pipelined=off  XmcBlockStatus=1  maskContainerNames=tabcontainer1  block_type=addsub  block_config=sysgen:Addsub_config
  AddSub2 : hdlBasic/AddSub  mode=Addition  use_carryin=off  use_carryout=off  en=off  latency=0  precision=User Defined  arith_type="Signed  (2's comp)"  n_bits=16  bin_pt=0  quantization="Round  (unbiased: +/- Inf)"  overflow=Flag as error  use_behavioral_HDL=off  hw_selection=Fabric  pipelined=off  XmcBlockStatus=1  maskContainerNames=tabcontainer1  block_type=addsub  block_config=sysgen:Addsub_config
  AddSub3 : hdlBasic/AddSub  mode=Subtraction  use_carryin=off  use_carryout=off  en=off  latency=0  precision=User Defined  arith_type="Signed  (2's comp)"  n_bits=16  bin_pt=0  quantization="Round  (unbiased: +/- Inf)"  overflow=Flag as error  use_behavioral_HDL=off  hw_selection=Fabric  pipelined=off  XmcBlockStatus=1  maskContainerNames=tabcontainer1  block_type=addsub  block_config=sysgen:Addsub_config
  AddSub4 : hdlBasic/AddSub  mode=Subtraction  use_carryin=off  use_carryout=off  en=off  latency=0  precision=User Defined  arith_type="Signed  (2's comp)"  n_bits=16  bin_pt=0  quantization="Round  (unbiased: +/- Inf)"  overflow=Flag as error  use_behavioral_HDL=off  hw_selection=Fabric  pipelined=off  XmcBlockStatus=1  maskContainerNames=tabcontainer1  block_type=addsub  block_config=sysgen:Addsub_config
  Delay2 : hdlBasic/Delay  rst=off  en=off  latency=7  reg_retiming=off  XmcBlockStatus=1  maskContainerNames=group1  block_type=delay  block_config=sysgen:Delay_config
  Delay3 : hdlBasic/Delay  rst=off  en=off  latency=7  reg_retiming=off  XmcBlockStatus=1  maskContainerNames=group1  block_type=delay  block_config=sysgen:Delay_config
  Out2_r : Outport
  Out2_i : Outport  Port=2
  Out1_r : Outport  Port=3
  Out1_i : Outport  Port=4
  wires:
  Delay3/1 -> Out2_i/1
  Delay2/1 -> Out2_r/1
  im1/1 -> AddSub3/2, AddSub1/2
  re1/1 -> AddSub4/2, AddSub2/2
  AddSub1/1 -> Delay3/1
  AddSub2/1 -> Delay2/1
  im2/1 -> AddSub3/1, AddSub1/1
  re2/1 -> AddSub4/1, AddSub2/1
  AddSub3/1 -> Out1_i/1
  AddSub4/1 -> Out1_r/1

== system sys1/SAR/stream/stream_fft/stage2/Multiplexer ==
  r1 : Inport
  i1 : Inport  Port=2
  r2 : Inport  Port=3
  i2 : Inport  Port=4
  cnt : Inport  Port=5
  BitBasher : hdlBasic/BitBasher  bitexpr=a={b[11]}  display_expr=off  sr_1=a  arith_type1=Unsigned  bin_pt1=0  sr_2=2  arith_type2=Unsigned  bin_pt2=0  sr_3=3  arith_type3=Unsigned  bin_pt3=0  sr_4=4  arith_type4=Unsigned  bin_pt4=0  XmcBlockStatus=1  maskContainerNames=group1  block_type=bitbasher  block_config=sysgen:BitBasher_config
  Inverter : hdlBasic/Inverter  en=off  latency=0  XmcBlockStatus=1  maskContainerNames=group2  block_type=inv  block_config=sysgen:Inverter_config
  Mux : hdlBasic/Mux  inputs=2  en=off  latency=0  precision=Full  arith_type=Unsigned  n_bits=16  bin_pt=14  quantization=Truncate  overflow=Wrap  XmcBlockStatus=1  maskContainerNames=tabcontainer1  block_type=mux  block_config=sysgen:Mux_config
  Mux1 : hdlBasic/Mux  inputs=2  en=off  latency=0  precision=Full  arith_type=Unsigned  n_bits=16  bin_pt=14  quantization=Truncate  overflow=Wrap  XmcBlockStatus=1  maskContainerNames=tabcontainer1  block_type=mux  block_config=sysgen:Mux_config
  rr : Outport
  ii : Outport  Port=2
  wires:
  Inverter/1 -> Mux1/1, Mux/1
  cnt/1 -> BitBasher/1
  Mux/1 -> rr/1
  Mux1/1 -> ii/1
  i1/1 -> Mux1/3
  r2/1 -> Mux/2
  BitBasher/1 -> Inverter/1
  i2/1 -> Mux1/2
  r1/1 -> Mux/3

== system sys1/SAR/stream/stream_fft/stage2/Twiddle ==
  r : Inport
  i : Inport  Port=2
  cnt : Inport  Port=3
  BitBasher1 : hdlBasic/BitBasher  bitexpr=a={b[10:10]}  display_expr=off  sr_1=a  arith_type1=Unsigned  bin_pt1=0  sr_2=2  arith_type2=Unsigned  bin_pt2=0  sr_3=3  arith_type3=Unsigned  bin_pt3=0  sr_4=4  arith_type4=Unsigned  bin_pt4=0  XmcBlockStatus=1  maskContainerNames=group1  block_type=bitbasher  block_config=sysgen:BitBasher_config
  Complex Multiplier 6.0 : hdlDSPIP/Complex Multiplier 6.0   hasatlast=off  hasatuser=off  atuserwidth=1  hasbtlast=off  hasbtuser=off  btuserwidth=1  multtype=Use_Mults  optimizegoal=Resources  flowcontrol=NonBlocking  outputwidth=32  roundmode=Truncate  hasctrltlast=off  hasctrltuser=off  ctrltuserwidth=1  outtlastbehv=Null  latencyconfig=Manual  minimumlatency=6  aclken=off  aresetn=off  trim_axipin_name=on  simulation_type=hybrid_sim  simulation_model=sysgen:cmpy_v6_0  data_path_portlist={ 's_axis_a_tdata_real', 's_axis_a_tdata_imag', 's_axis_b_tdata_real', 's_axis_b_tdata_imag', 's_axis_ctrl_tdata_rounding_bit', 'm_axis_dout_tdata_real', 'm_axis_dout_tdata_imag' }  aportwidth=63  bportwidth=63  ip_name=Complex Multiplier  ip_version=6.0  dsptool_ready=true  ipcore_usecache=true  ipcore_useipmodelcache=true  ipcore_verbose=false  ipcore_latency_parameter='minimumlatency'  wrapper_available=true  port_translation_map={ 'aclken' => 'en', 'aresetn' => 'rst'}  XmcBlockStatus=1  maskContainerNames=tabcontainer1  block_type=cmpy_v6_0  block_config=sysgen:rodinimport_config
  Constant2 : hdlBasic/Constant  const=1  gui_display_data_type=Boolean  arith_type=Boolean  n_bits=16  bin_pt=14  preci_type=Single  exp_width=8  frac_width=24  explicit_period=on  period=ts  XmcBlockStatus=1  maskContainerNames=tabcontainer1  block_type=constant  block_config=sysgen:Constant_config
  Constant3 : hdlBasic/Constant  const=1  gui_display_data_type=Boolean  arith_type=Boolean  n_bits=16  bin_pt=14  preci_type=Single  exp_width=8  frac_width=24  explicit_period=on  period=ts  XmcBlockStatus=1  maskContainerNames=tabcontainer1  block_type=constant  block_config=sysgen:Constant_config
  Convert1 : hdlBasic/Convert  gui_display_data_type=Fixed-point  arith_type=Signed (2's comp)  n_bits=16  bin_pt=0  float_type=Single  exp_bits=8  fraction_bits=24  quantization=Truncate  overflow=Flag as error  en=off  latency=0  pipeline=off  XmcBlockStatus=1  maskContainerNames=group2  block_type=convert  block_config=sysgen:Convert_config  block_width=595  block_height=885
  Convert2 : hdlBasic/Convert  gui_display_data_type=Fixed-point  arith_type=Signed (2's comp)  n_bits=16  bin_pt=0  float_type=Single  exp_bits=8  fraction_bits=24  quantization=Truncate  overflow=Flag as error  en=off  latency=0  pipeline=off  XmcBlockStatus=1  maskContainerNames=group2  block_type=convert  block_config=sysgen:Convert_config  block_width=595  block_height=885
  Delay2 : hdlBasic/Delay  rst=off  en=off  latency=1  reg_retiming=off  XmcBlockStatus=1  maskContainerNames=group1  block_type=delay  block_config=sysgen:Delay_config
  Delay3 : hdlBasic/Delay  rst=off  en=off  latency=1  reg_retiming=off  XmcBlockStatus=1  maskContainerNames=group1  block_type=delay  block_config=sysgen:Delay_config
  ROM : hdlBasic/ROM  depth=length(w2)  initVector=real(w2)  distributed_mem=Block RAM  rst=off  init_reg=0  en=off  latency=1  gui_display_data_type=Fixed-point  arith_type="Signed  (2's comp)"  n_bits=16  bin_pt=15  preci_type=Single  exp_width=8  frac_width=24  optimize=Area  use_rpm=on  simulation_type=fast_sim  XmcBlockStatus=1  maskContainerNames=tabcontainer1  block_type=sprom  block_config=sysgen:SPROM_config
  ROM1 : hdlBasic/ROM  depth=length(w2)  initVector=imag(w2)  distributed_mem=Block RAM  rst=off  init_reg=0  en=off  latency=1  gui_display_data_type=Fixed-point  arith_type="Signed  (2's comp)"  n_bits=16  bin_pt=15  preci_type=Single  exp_width=8  frac_width=24  optimize=Area  use_rpm=on  simulation_type=fast_sim  XmcBlockStatus=1  maskContainerNames=tabcontainer1  block_type=sprom  block_config=sysgen:SPROM_config
  rr : Outport
  ii : Outport  Port=2
  wires:
  Delay3/1 -> Complex Multiplier 6.0/3
  Delay2/1 -> Complex Multiplier 6.0/2
  Convert1/1 -> rr/1
  Convert2/1 -> ii/1
  cnt/1 -> BitBasher1/1
  r/1 -> Delay3/1
  Complex Multiplier 6.0/3 -> Convert1/1
  i/1 -> Delay2/1
  Constant3/1 -> Complex Multiplier 6.0/4
  ROM/1 -> Complex Multiplier 6.0/6
  Constant2/1 -> Complex Multiplier 6.0/1
  Complex Multiplier 6.0/2 -> Convert2/1
  BitBasher1/1 -> ROM1/1, ROM/1
  ROM1/1 -> Complex Multiplier 6.0/5

== system sys1/SAR/stream/stream_fft/stage2/delay ==
  r : Inport
  i : Inport  Port=2
  cnt : Inport  Port=3
  r1 : Inport  Port=4
  i1 : Inport  Port=5
  BitBasher : hdlBasic/BitBasher  bitexpr=a={b[11]}  display_expr=off  sr_1=a  arith_type1=Unsigned  bin_pt1=0  sr_2=2  arith_type2=Unsigned  bin_pt2=0  sr_3=3  arith_type3=Unsigned  bin_pt3=0  sr_4=4  arith_type4=Unsigned  bin_pt4=0  XmcBlockStatus=1  maskContainerNames=group1  block_type=bitbasher  block_config=sysgen:BitBasher_config
  Inverter : hdlBasic/Inverter  en=off  latency=0  XmcBlockStatus=1  maskContainerNames=group2  block_type=inv  block_config=sysgen:Inverter_config
  Mux : hdlBasic/Mux  inputs=2  en=off  latency=0  precision=Full  arith_type=Unsigned  n_bits=16  bin_pt=14  quantization=Truncate  overflow=Wrap  XmcBlockStatus=1  maskContainerNames=tabcontainer1  block_type=mux  block_config=sysgen:Mux_config
  Mux1 : hdlBasic/Mux  inputs=2  en=off  latency=0  precision=Full  arith_type=Unsigned  n_bits=16  bin_pt=14  quantization=Truncate  overflow=Wrap  XmcBlockStatus=1  maskContainerNames=tabcontainer1  block_type=mux  block_config=sysgen:Mux_config
  delay : Subsystem
  delay1 : Subsystem
  rr : Outport
  ii : Outport  Port=2
  wires:
  i/1 -> Mux1/3
  r/1 -> Mux/3
  delay1/1(out) -> ii/1
  delay/1(out) -> rr/1
  i1/1 -> Mux1/2
  r1/1 -> Mux/2
  Mux1/1 -> delay1/1(in)
  Mux/1 -> delay/1(in)
  BitBasher/1 -> Inverter/1
  cnt/1 -> BitBasher/1
  Inverter/1 -> Mux/1, Mux1/1

== system sys1/SAR/stream/stream_fft/stage3/BF ==
  re2 : Inport
  im2 : Inport  Port=2
  re1 : Inport  Port=3
  im1 : Inport  Port=4
  AddSub1 : hdlBasic/AddSub  mode=Addition  use_carryin=off  use_carryout=off  en=off  latency=0  precision=User Defined  arith_type="Signed  (2's comp)"  n_bits=16  bin_pt=0  quantization="Round  (unbiased: +/- Inf)"  overflow=Flag as error  use_behavioral_HDL=off  hw_selection=Fabric  pipelined=off  XmcBlockStatus=1  maskContainerNames=tabcontainer1  block_type=addsub  block_config=sysgen:Addsub_config
  AddSub2 : hdlBasic/AddSub  mode=Addition  use_carryin=off  use_carryout=off  en=off  latency=0  precision=User Defined  arith_type="Signed  (2's comp)"  n_bits=16  bin_pt=0  quantization="Round  (unbiased: +/- Inf)"  overflow=Flag as error  use_behavioral_HDL=off  hw_selection=Fabric  pipelined=off  XmcBlockStatus=1  maskContainerNames=tabcontainer1  block_type=addsub  block_config=sysgen:Addsub_config
  AddSub3 : hdlBasic/AddSub  mode=Subtraction  use_carryin=off  use_carryout=off  en=off  latency=0  precision=User Defined  arith_type="Signed  (2's comp)"  n_bits=16  bin_pt=0  quantization="Round  (unbiased: +/- Inf)"  overflow=Flag as error  use_behavioral_HDL=off  hw_selection=Fabric  pipelined=off  XmcBlockStatus=1  maskContainerNames=tabcontainer1  block_type=addsub  block_config=sysgen:Addsub_config
  AddSub4 : hdlBasic/AddSub  mode=Subtraction  use_carryin=off  use_carryout=off  en=off  latency=0  precision=User Defined  arith_type="Signed  (2's comp)"  n_bits=16  bin_pt=0  quantization="Round  (unbiased: +/- Inf)"  overflow=Flag as error  use_behavioral_HDL=off  hw_selection=Fabric  pipelined=off  XmcBlockStatus=1  maskContainerNames=tabcontainer1  block_type=addsub  block_config=sysgen:Addsub_config
  Delay2 : hdlBasic/Delay  rst=off  en=off  latency=7  reg_retiming=off  XmcBlockStatus=1  maskContainerNames=group1  block_type=delay  block_config=sysgen:Delay_config
  Delay3 : hdlBasic/Delay  rst=off  en=off  latency=7  reg_retiming=off  XmcBlockStatus=1  maskContainerNames=group1  block_type=delay  block_config=sysgen:Delay_config
  Out2_r : Outport
  Out2_i : Outport  Port=2
  Out1_r : Outport  Port=3
  Out1_i : Outport  Port=4
  wires:
  AddSub4/1 -> Out1_r/1
  AddSub3/1 -> Out1_i/1
  re2/1 -> AddSub2/1, AddSub4/1
  im2/1 -> AddSub1/1, AddSub3/1
  AddSub2/1 -> Delay2/1
  AddSub1/1 -> Delay3/1
  re1/1 -> AddSub2/2, AddSub4/2
  im1/1 -> AddSub1/2, AddSub3/2
  Delay2/1 -> Out2_r/1
  Delay3/1 -> Out2_i/1
